simulink library "boatModels"  (R2024b)
settings: Solver=VariableStepAuto  StartTime=0.0  StopTime=10.0  RelTol=1e-3
values from neighbouring files (symbols this model uses):
  boat = setupBoat()    [boatMain.m]    (also in main.m; scheduled_main.m)
libraries: sharedtransform x1
settings Model: Creator=domac  LastModifiedBy=domac

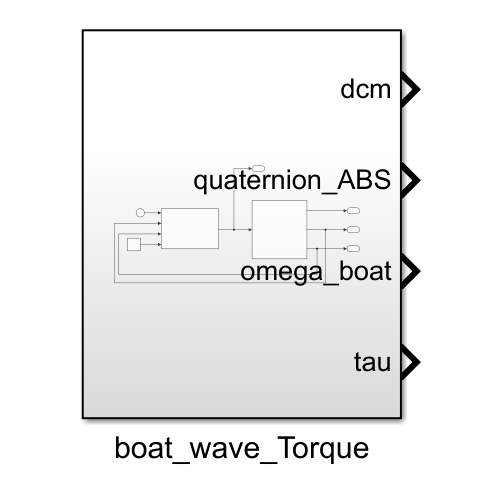
[thumbnail: Simulink's stored preview of the top-level diagram]
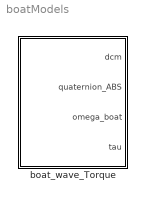
== system boatModels ==
  boat_wave_Torque : Subsystem

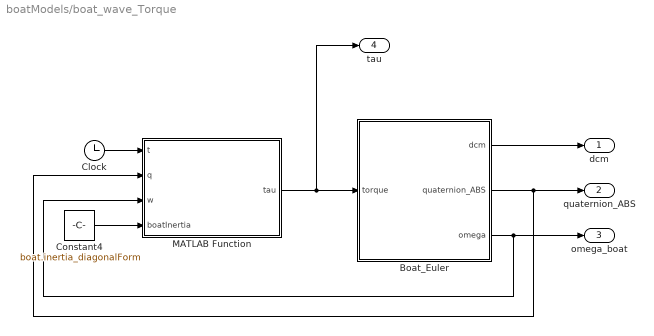
== system boatModels/boat_wave_Torque ==
  Boat_Euler : Subsystem
  Clock : Clock
  Constant4 : Constant  Value=boat.inertia_diagonalForm
  MATLAB Function : MATLAB Function  TreatAsAtomicUnit=on
  dcm : Outport
  quaternion_ABS : Outport  Port=2
  omega_boat : Outport  Port=3
  tau : Outport  Port=4
  wires:
  MATLAB Function/1(tau) -> tau/1, Boat_Euler/1(torque)
  Boat_Euler/3(omega) -> omega_boat/1, MATLAB Function/3(w)
  Constant4/1 -> MATLAB Function/4(boatInertia)
  Boat_Euler/2(quaternion_ABS) -> quaternion_ABS/1, MATLAB Function/2(q)
  Clock/1 -> MATLAB Function/1(t)
  Boat_Euler/1(dcm) -> dcm/1

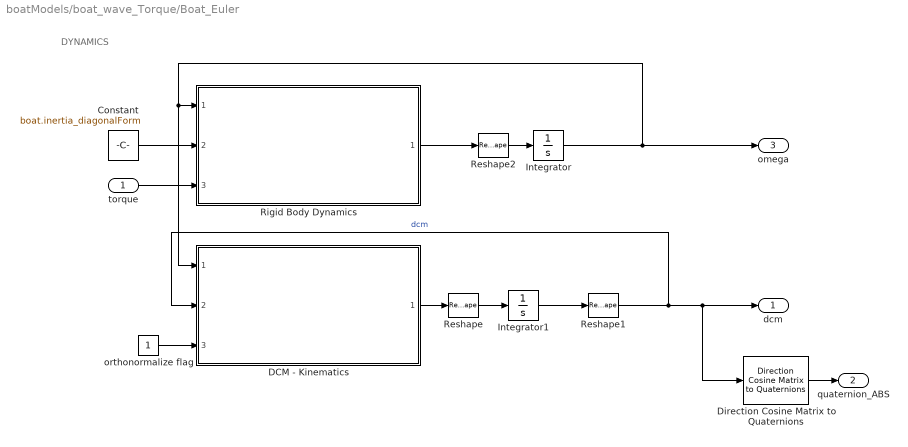
== system boatModels/boat_wave_Torque/Boat_Euler ==
  note: DYNAMICS
  torque : Inport
  " DCM - Kinematics" : Subsystem  ReferencedSubsystem=Kinematics
  Constant : Constant  Value=boat.inertia_diagonalForm  VectorParams1D=off
  Direction Cosine Matrix to Quaternions : sharedtransform/Direction Cosine Matrix  to Quaternions  aMode=0  action=None  tolerance=eps(2)
  Integrator : Integrator  InitialCondition=boat.w0
  Integrator1 : Integrator  InitialCondition=[boat.initialDCM(:,1); boat.initialDCM(:,2); boat.initialDCM(:,3)]
  Reshape : Reshape  OutputDimensionality=Column vector (2-D)
  Reshape1 : Reshape  OutputDimensionality=Customize  OutputDimensions=[3, 3]
  Reshape2 : Reshape  OutputDimensionality=Column vector (2-D)
  Rigid Body Dynamics : Subsystem  ReferencedSubsystem=Dynamics
  orthonormalize flag : Constant
  dcm : Outport
  quaternion_ABS : Outport  Port=2
  omega : Outport  Port=3
  wires:
  orthonormalize flag/1 -> " DCM - Kinematics"/3
  Reshape/1 -> Integrator1/1
  Integrator1/1 -> Reshape1/1
  Rigid Body Dynamics/1 -> Reshape2/1
  Constant/1 -> Rigid Body Dynamics/2
  " DCM - Kinematics"/1 -> Reshape/1
  Integrator/1 -> omega/1, " DCM - Kinematics"/1, Rigid Body Dynamics/1
  Reshape2/1 -> Integrator/1
  Reshape1/1 -> Direction Cosine Matrix to Quaternions/1, dcm/1, " DCM - Kinematics"/2  "dcm"
  torque/1 -> Rigid Body Dynamics/3
  Direction Cosine Matrix to Quaternions/1 -> quaternion_ABS/1

== matlab function boatModels/boat_wave_Torque/MATLAB Function ==
  data: t input; tau output; q input; w input; boatInertia input
function tau = waveTorque(t, q, w, boatInertia)
q = q / norm(q);
q0 = q(1); q1 = q(2); q2 = q(3); q3 = q(4);
phi   = atan2(2*(q0*q1 + q2*q3), 1 - 2*(q1^2 + q2^2));
theta = asin(max(-1, min(1, 2*(q0*q2 - q3*q1))));
psi   = atan2(2*(q0*q3 + q1*q2), 1 - 2*(q2^2 + q3^2));

% boat
rho = 1025; g = 9.81;
Vol = 2.0;  GMT = 0.8;  GML = 6.0;
Ixx = boatInertia(1);  Iyy = boatInertia(2);
zr = 0.10;  zp = 0.25;  Bz = 500;

% sea parameters
Hs = 1.0; Tp = 6; gam = 3.3;
chi = 90*pi/180;     
N = 50;

Cphi = rho*g*Vol*GMT;  Cth = rho*g*Vol*GML;
Bphi = 2*zr*sqrt(Cphi*Ixx);  Bth = 2*zp*sqrt(Cth*Iyy);

wp = 2*pi/Tp; wmin = 0.5*wp; wmax = 3*wp; dw = (wmax-wmin)/N;
i = (1:N)';
wi = wmin + (i - 1 + mod(i*0.6180339887,1))*dw;
sig = 0.07 + 0.02*(wi > wp);
S = (5/16)*Hs^2*wp^4./wi.^5 .* exp(-1.25*(wp./wi).^4) ...
    .* gam.^exp(-(wi-wp).^2./(2*sig.^2*wp^2)) * (1-0.287*log(gam));
kai   = (wi.^2/g) .* sqrt(2*S*dw);
phi_i = mod(i*2.399963229728653, 2*pi);

alpha = sum(kai .* sin(wi*t + phi_i));
beta  = chi - psi;

tau = [ -Cphi*(phi   - sin(beta)*alpha) - Bphi*w(1);
        -Cth *(theta - cos(beta)*alpha) - Bth *w(2);
        -Bz*w(3) ];

tau = tau * 50;

end
